simulink model "HVDC_Simu"  (R2023b)
settings: Solver=VariableStepAuto  StartTime=0.0  StopTime=0.08  RelTol=1e-3
libraries: spsDiodeLib x6, spsMultimeterLib x5, spsACVoltageSourceLib x3, spsRMSLib x3, spsSeriesRLCBranchLib x2, spsGroundLib x2, spsThreePhaseTransformerTwoWindingsLib x1, spsThreePhaseVIMeasurementLib x1, sps_lib x1
settings Model: Creator=ASUS  LastModifiedBy=ASUS

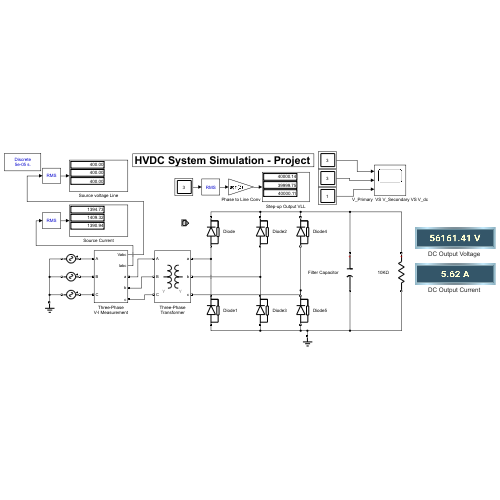
[thumbnail: Simulink's stored preview of the top-level diagram]
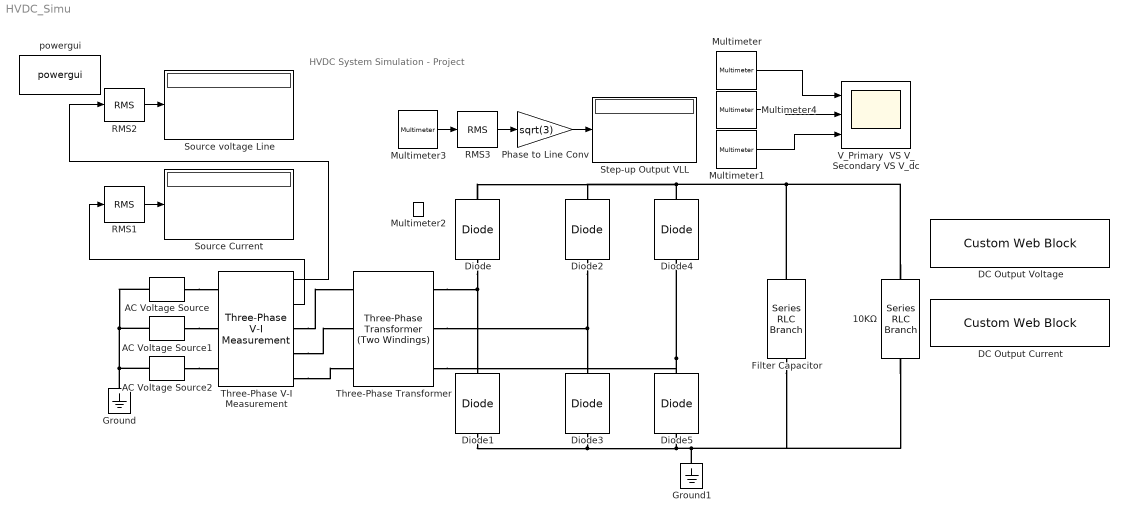
== system HVDC_Simu ==
  note: HVDC System Simulation - Project
  "10KΩ " : spsSeriesRLCBranchLib/Series RLC Branch  LConnTagsString=__new0  RConnTagsString=__new0  BranchType=R  Resistance=10000  Inductance=1e-3  SetiL0=off  InitialCurrent=0  Capacitance=1e-6  Setx0=off  InitialVoltage=0  Measurements=Branch voltage and current
  AC Voltage Source : spsACVoltageSourceLib/AC Voltage Source  Amplitude=(400/sqrt(3))*sqrt(2)  Phase=0  Frequency=60  SampleTime=0  Measurements=Voltage  BusType=swing  Pref=10e3  Qref=0  Qmin=-inf  Qmax=+inf
  AC Voltage Source1 : spsACVoltageSourceLib/AC Voltage Source  Amplitude=(400/sqrt(3))*sqrt(2)  Phase=120  Frequency=60  SampleTime=0  Measurements=Voltage  BusType=swing  Pref=10e3  Qref=0  Qmin=-inf  Qmax=+inf
  AC Voltage Source2 : spsACVoltageSourceLib/AC Voltage Source  Amplitude=(400/sqrt(3))*sqrt(2)  Phase=240  Frequency=60  SampleTime=0  Measurements=Voltage  BusType=swing  Pref=10e3  Qref=0  Qmin=-inf  Qmax=+inf
  "DC Output Current " : CustomWebBlock  LabelPosition=Hide  ShowInitialText=on  Configuration="{\"components\":[{\"name\":\"DisplayComponent\",\"settings\":{\"bold\":true,\"font\":\"Roboto\",\"fontColor\":[255,255,200],\"fontSize\":\"22\",\"format\":\"Custom\",\"formatString\":\"%.2f A\",\"italic\":false,\"position\":[0,0,1,1],\"underline\":false}},{\"name\":\"BackgroundImageComponent\",\"settings\":{\"image\":{\"size\":[300,80],\"src\":\"data:image\\/svg+xml;base64,PHN2ZyBpZD0iZnJhbWUiIHhtbG5zPSJodHRwOi8vd3d3LnczLm9yZy8yMDAwL3N2ZyIgeG1sbnM6eGxpbms9Imh0dHA6Ly93d3cudzMub3JnLzE5OTkveGxpbmsiIHZpZXdCb3g9IjAgMCAzODAgMTAxIj48ZGVmcz48c3R5bGU+LmNscy0xe2ZpbGw6IzAwMmI0Mjt9LmNscy0ye2ZpbGw6IzQyNzA4Mjt9LmNscy0ze2ZpbGw6dXJsKCNyYWRpYWwtZ3JhZGllbnQpO308L3N0eWxlPjxyYWRpYWxHcmFkaWVudCBpZD0icmFkaWFsLWdyYWRpZW50IiBjeD0iMTkwIiBjeT0iNTAuNSIgcj0iMjY5LjIxIiBncmFkaWVudFVuaXRzPSJ1c2VyU3BhY2VPblVzZSI+PHN0b3Agb2Zmc2V0PSIwLjAxIiBzdG9wLWNvbG9yPSIjM2U0ZjU4Ii8+PHN0b3Agb2Zmc2V0PSIwLjA2IiBzdG9wLWNvbG9yPSIjNDQ1NzYxIi8+PHN0b3Agb2Zmc2V0PSIwLjE1IiBzdG9wLWNvbG9yPSIjNTU2YTc2Ii8+PHN0b3Agb2Zmc2V0PSIwLjI1IiBzdG9wLWNvbG9yPSIjNmQ4ODk1Ii8+PHN0b3Agb2Zmc2V0PSIwLjM4IiBzdG9wLWNvbG9yPSIjOGZiMmMzIi8+PHN0b3Agb2Zmc2V0PSIwLjUyIiBzdG9wLWNvbG9yPSIjYjZlNGZhIi8+PHN0b3Agb2Zmc2V0PSIxIiBzdG9wLWNvbG9yPSIjMTU0NjU3Ii8+PC9yYWRpYWxHcmFkaWVudD48L2RlZnM+PGcgaWQ9IkxheWVyXzIiIGRhdGEtbmFtZT0iTGF5ZXIgMiI+PGcgaWQ9IkxheWVyXzEtMiIgZGF0YS1uYW1lPSJMYXllciAxLTIiPjxyZWN0IGlkPSJyZWN0MTAzNiIgY2xhc3M9ImNscy0xIiB4PSIxMSIgeT0iMTEiIHdpZHRoPSIzNTgiIGhlaWdodD0iNzkiLz48cGF0aCBpZD0icGF0aDEwMzgiIGNsYXNzPSJjbHMtMiIgZD0iTTgsOFY5M0gzNzJWOFpNMzY5LDkwSDExVjExSDM2OVoiLz48cGF0aCBpZD0icGF0aDEwNDAiIGNsYXNzPSJjbHMtMyIgZD0iTTAsMFYxMDFIMzgwVjBaTTM3Miw5M0g4VjhIMzcyWiIvPjwvZz48L2c+PC9zdmc+\",\"srcOrientation\":\"Right\"},\"position\":[0,0,1,1],\"scaleMode\":\"0\"}},{\"name\":\"ForegroundImageComponent\",\"settings\":{\"angle\":0,\"image\":{\"size\":[0,0],\"src\":\"default\"},\"isForeground\":1,\"position\":[0,0,1,1],\"scaleMode\":\"0\"}}],\"settings\":{\"BindingType\":\"signal\",\"aspectRatio\":1.032258064516129,\"backgroundColor\":[0,0,0,\"1\"],\"backgroundOffset\":0.14,\"backgroundOpacity\":1,\"fixedAspectRatio\":\"on\",\"showBackgroundColor\":false,\"value\":0,\"version\":\"R2023b\"},\"type\":\"Display\"}"
  "DC Output Voltage " : CustomWebBlock  LabelPosition=Hide  ShowInitialText=on  Configuration="{\"components\":[{\"name\":\"DisplayComponent\",\"settings\":{\"bold\":true,\"font\":\"Roboto\",\"fontColor\":[255,255,200],\"fontSize\":\"22\",\"format\":\"Custom\",\"formatString\":\"%.2f V\",\"italic\":false,\"position\":[0,0,1,1],\"underline\":false}},{\"name\":\"BackgroundImageComponent\",\"settings\":{\"image\":{\"size\":[300,80],\"src\":\"data:image\\/svg+xml;base64,PHN2ZyBpZD0iZnJhbWUiIHhtbG5zPSJodHRwOi8vd3d3LnczLm9yZy8yMDAwL3N2ZyIgeG1sbnM6eGxpbms9Imh0dHA6Ly93d3cudzMub3JnLzE5OTkveGxpbmsiIHZpZXdCb3g9IjAgMCAzODAgMTAxIj48ZGVmcz48c3R5bGU+LmNscy0xe2ZpbGw6IzAwMmI0Mjt9LmNscy0ye2ZpbGw6IzQyNzA4Mjt9LmNscy0ze2ZpbGw6dXJsKCNyYWRpYWwtZ3JhZGllbnQpO308L3N0eWxlPjxyYWRpYWxHcmFkaWVudCBpZD0icmFkaWFsLWdyYWRpZW50IiBjeD0iMTkwIiBjeT0iNTAuNSIgcj0iMjY5LjIxIiBncmFkaWVudFVuaXRzPSJ1c2VyU3BhY2VPblVzZSI+PHN0b3Agb2Zmc2V0PSIwLjAxIiBzdG9wLWNvbG9yPSIjM2U0ZjU4Ii8+PHN0b3Agb2Zmc2V0PSIwLjA2IiBzdG9wLWNvbG9yPSIjNDQ1NzYxIi8+PHN0b3Agb2Zmc2V0PSIwLjE1IiBzdG9wLWNvbG9yPSIjNTU2YTc2Ii8+PHN0b3Agb2Zmc2V0PSIwLjI1IiBzdG9wLWNvbG9yPSIjNmQ4ODk1Ii8+PHN0b3Agb2Zmc2V0PSIwLjM4IiBzdG9wLWNvbG9yPSIjOGZiMmMzIi8+PHN0b3Agb2Zmc2V0PSIwLjUyIiBzdG9wLWNvbG9yPSIjYjZlNGZhIi8+PHN0b3Agb2Zmc2V0PSIxIiBzdG9wLWNvbG9yPSIjMTU0NjU3Ii8+PC9yYWRpYWxHcmFkaWVudD48L2RlZnM+PGcgaWQ9IkxheWVyXzIiIGRhdGEtbmFtZT0iTGF5ZXIgMiI+PGcgaWQ9IkxheWVyXzEtMiIgZGF0YS1uYW1lPSJMYXllciAxLTIiPjxyZWN0IGlkPSJyZWN0MTAzNiIgY2xhc3M9ImNscy0xIiB4PSIxMSIgeT0iMTEiIHdpZHRoPSIzNTgiIGhlaWdodD0iNzkiLz48cGF0aCBpZD0icGF0aDEwMzgiIGNsYXNzPSJjbHMtMiIgZD0iTTgsOFY5M0gzNzJWOFpNMzY5LDkwSDExVjExSDM2OVoiLz48cGF0aCBpZD0icGF0aDEwNDAiIGNsYXNzPSJjbHMtMyIgZD0iTTAsMFYxMDFIMzgwVjBaTTM3Miw5M0g4VjhIMzcyWiIvPjwvZz48L2c+PC9zdmc+\",\"srcOrientation\":\"Right\"},\"position\":[0,0,1,1],\"scaleMode\":\"0\"}},{\"name\":\"ForegroundImageComponent\",\"settings\":{\"angle\":0,\"image\":{\"size\":[0,0],\"src\":\"default\"},\"isForeground\":1,\"position\":[0,0,1,1],\"scaleMode\":\"0\"}}],\"settings\":{\"BindingType\":\"signal\",\"aspectRatio\":1.032258064516129,\"backgroundColor\":[0,0,0,\"1\"],\"backgroundOffset\":0.14,\"backgroundOpacity\":1,\"fixedAspectRatio\":\"on\",\"showBackgroundColor\":false,\"value\":0,\"version\":\"R2023b\"},\"type\":\"Display\"}"
  Diode{,1..5} (6 alike) : spsDiodeLib/Diode  Ron=0.001  Lon=0  Vf=0.8  IC=0  UseSnubber=0  Rs=500  Cs=250e-9  Measurements=off
  Filter Capacitor : spsSeriesRLCBranchLib/Series RLC Branch  LConnTagsString=__new0  RConnTagsString=__new0  BranchType=C  Resistance=10000  Inductance=1e-3  SetiL0=off  InitialCurrent=0  Capacitance=20e-6  Setx0=on  InitialVoltage=56571  Measurements=Branch voltage and current
  Ground : spsGroundLib/Ground  LConnTagsString=a
  Ground1 : spsGroundLib/Ground  LConnTagsString=a
  Multimeter : spsMultimeterLib/Multimeter  L=28  sel=[9 10 11]  yselected={}  Gain=[1 1 1]  OutputType=Complex  PlotAtSimulationStop=off  PhasorSimulation=off
  Multimeter1 : spsMultimeterLib/Multimeter  L=28  sel=1  yselected={}  Gain=1  OutputType=Complex  PlotAtSimulationStop=on  PhasorSimulation=off
  Multimeter2 : spsMultimeterLib/Multimeter  L=28  sel=12  yselected={}  Gain=1  OutputType=Complex  PlotAtSimulationStop=off  PhasorSimulation=off
  Multimeter3 : spsMultimeterLib/Multimeter  L=28  sel=[6 7 8]  yselected={}  Gain=[1 1 1]  OutputType=Complex  PlotAtSimulationStop=on  PhasorSimulation=off
  Multimeter4 : spsMultimeterLib/Multimeter  L=28  sel=[6 7 8]  yselected={}  Gain=[1 1 1]  OutputType=Complex  PlotAtSimulationStop=on  PhasorSimulation=off
  Phase to Line Conv : Gain  Gain=sqrt(3)
  RMS1 : spsRMSLib/RMS  TrueRMS=on  Freq=60  RMSInit=120  Ts=0
  RMS2 : spsRMSLib/RMS  TrueRMS=on  Freq=60  RMSInit=120  Ts=0
  RMS3 : spsRMSLib/RMS  TrueRMS=on  Freq=60  RMSInit=120  Ts=0
  Source Current : Display
      settings: Format=bank
  Source voltage Line : Display
      settings: Format=bank
  Step-up Output VLL : Display
      settings: Format=bank
  "Three-Phase Transformer " : spsThreePhaseTransformerTwoWindingsLib/Three-Phase Transformer (Two Windings)  Winding1Connection=Y  Winding2Connection=Y  CoreType=Three single-phase transformers  SetSaturation=off  Hysteresis=off  DataFile='hysteresis'  SetInitialFlux=off  Measurements=All measurements (V I Fluxes)  UNITS=SI  NominalPower=[ 50e3 , 60 ]  Winding1=[400/sqrt(3) 0 0]  Winding2=[40e3/sqrt(3) 0 0]  Rm=inf  Lm=inf  L0=0.5  Saturation=[0 0;0.66653 1910.3;277.72 2419.7]  InitialFluxes=[ 0.8 , -0.8 , 0.7 ]  BreakLoop=off  DiscreteSolver=Trapezoidal iterative  DataType=on  TransfoNumber=1
  Three-Phase V-I Measurement : spsThreePhaseVIMeasurementLib/Three-Phase V-I Measurement  VoltageMeasurement=phase-to-phase  SetLabelV=off  LabelV=Vabc  Vpu=off  VpuLL=off  CurrentMeasurement=yes  SetLabelI=off  LabelI=Iabc  Ipu=off  Pbase=100e6  Vbase=500e3  OutputType=Complex  PhasorSimulation=off  PSBequivalent=0
  V_Primary  VS V_Secondary VS V_dc : Scope  NumInputPorts=3
  powergui : sps_lib/powergui  Priority=1  SimulationMode=Discrete  SampleTime=50e-6  frequency=60  Iterations=50  frequencyindice=60  Pbase=100e6  ErrMax=1e-4  UnitsV=kV  UnitsW=MW  buscounter=0  FunctionMessages=off  echomessages=off  EnableUseOfTLC=off  CurrentSourceSwitches=off  DisableSnubberDevices=off  DisableRonSwitches=off  DisableVfSwitches=off  DisplayEquations=off  AutomaticDiscreteSolvers=off  SolverType=Tustin/Backward Euler (TBE)  Interpol=off  ExternalGateDelay=off  methode=off  Ts=100  x0status=blocks  SPID=on  SwTol=0  HookPort=off  NonlinearTolerance=1e-4  nMaxIteration=100  ContinueOnMaxIteration=off  RestoreLinks=warning  ResistiveCurrentMeasurement=off  Frange=[0:2:500]  Ylog=off  Xlog=on  ShowGrid=off  save=off  variable=ZData  structure=0  ZoomFFT=off  StartTime=0.0  cycles=1  DisplayStyle=1  fundamental=60  FreqAxis=off  MaxFrequency=1000  frequencyindicesteady=1  RmsSteady=1  display=off
  wires:
  Three-Phase V-I Measurement/1 -> RMS2/1
  RMS2/1 -> Source voltage Line/1
  RMS1/1 -> Source Current/1
  Three-Phase V-I Measurement/2 -> RMS1/1
  Multimeter/1 -> V_Primary  VS V_Secondary VS V_dc/1
  Multimeter3/1 -> RMS3/1
  RMS3/1 -> Phase to Line Conv/1
  Phase to Line Conv/1 -> Step-up Output VLL/1
  Multimeter4/1 -> V_Primary  VS V_Secondary VS V_dc/2
  Multimeter1/1 -> V_Primary  VS V_Secondary VS V_dc/3
  connections:
  Ground/LConn1 -- AC Voltage Source2/LConn1 -- AC Voltage Source1/LConn1 -- AC Voltage Source/LConn1
  AC Voltage Source1/RConn1 -- Three-Phase V-I Measurement/LConn2
  AC Voltage Source2/RConn1 -- Three-Phase V-I Measurement/LConn3
  Three-Phase V-I Measurement/RConn1 -- "Three-Phase Transformer "/LConn1
  Three-Phase V-I Measurement/RConn2 -- "Three-Phase Transformer "/LConn2
  Three-Phase V-I Measurement/RConn3 -- "Three-Phase Transformer "/LConn3
  AC Voltage Source/RConn1 -- Three-Phase V-I Measurement/LConn1
  Diode/LConn1 -- "Three-Phase Transformer "/RConn1 -- Diode1/RConn1
  Diode2/LConn1 -- "Three-Phase Transformer "/RConn2 -- Diode3/RConn1
  Diode5/RConn1 -- Diode4/LConn1 -- "Three-Phase Transformer "/RConn3
  "10KΩ "/LConn1 -- Diode4/RConn1 -- Diode/RConn1 -- Diode2/RConn1 -- Filter Capacitor/LConn1
  Diode1/LConn1 -- "10KΩ "/RConn1 -- Filter Capacitor/RConn1 -- Ground1/LConn1 -- Diode5/LConn1 -- Diode3/LConn1
